simulink model "hw4_1"  (R2025a)
settings: Solver=VariableStepAuto  StartTime=0.0  StopTime=10  RelTol=1e-3
undefined symbols (not defined in the file): Kd, Ki, Kp
settings Model: Creator=BCC  LastModifiedBy=BCC

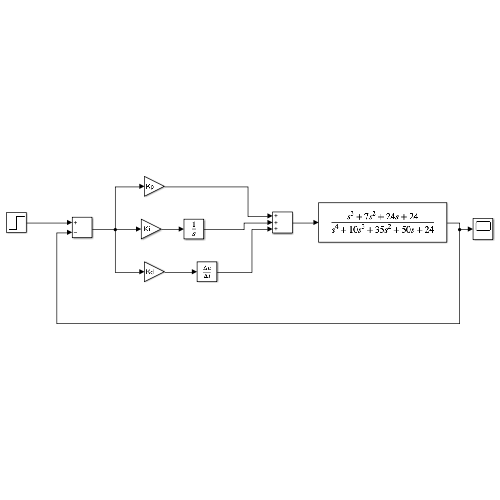
[thumbnail: Simulink's stored preview of the top-level diagram]
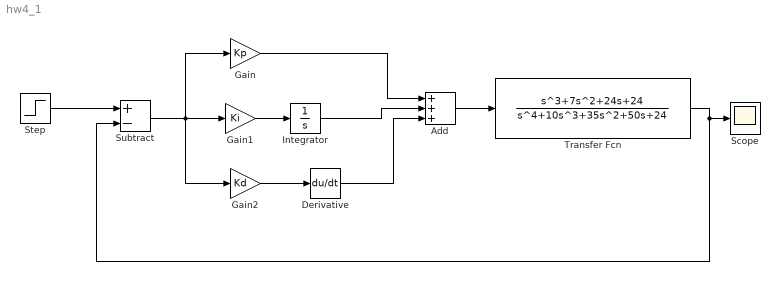
== system hw4_1 ==
  Add : Sum  Inputs=+++
  Derivative : Derivative
  Gain : Gain  Gain=Kp
  Gain1 : Gain  Gain=Ki
  Gain2 : Gain  Gain=Kd
  Integrator : Integrator
  Scope : Scope
      settings: ActiveDisplayYMinimum=-0.1421178706887144  ActiveDisplayYMaximum=1.27906083619843
  Step : Step  SampleTime=0
  Subtract : Sum  Inputs=+-
  Transfer Fcn : TransferFcn  Numerator=[1 7 24 24]  Denominator=[1 10 35 50 24]
  wires:
  Step/1 -> Subtract/1
  Transfer Fcn/1 -> Subtract/2, Scope/1
  Integrator/1 -> Add/2
  Subtract/1 -> Gain/1, Gain1/1, Gain2/1
  Gain/1 -> Add/1
  Gain2/1 -> Derivative/1
  Add/1 -> Transfer Fcn/1
  Gain1/1 -> Integrator/1
  Derivative/1 -> Add/3
